simulink subsystem "saturation"  (R2024b)
settings: Solver=VariableStepAuto  StartTime=0.0  StopTime=10.0  RelTol=1e-3
settings Model: Creator=pierb  LastModifiedBy=pierb

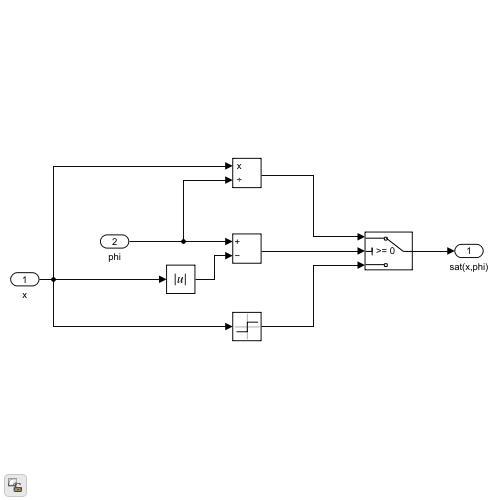
[thumbnail: Simulink's stored preview of the top-level diagram]
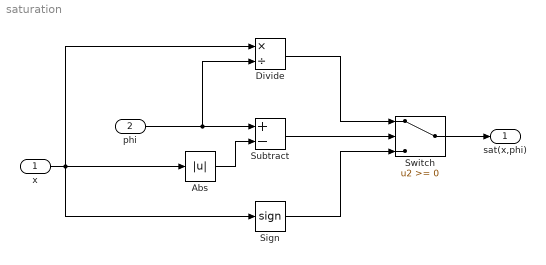
== system saturation ==
  x : Inport
  phi : Inport  Port=2
  Abs : Abs  SaturateOnIntegerOverflow=off
  Divide : Product  Inputs=*/
  Sign : Signum
  Subtract : Sum  Inputs=+-
  Switch : Switch  SaturateOnIntegerOverflow=off  InputSameDT=off
  sat(x,phi) : Outport
  wires:
  Switch/1 -> sat(x,phi)/1
  phi/1 -> Subtract/1, Divide/2
  x/1 -> Abs/1, Divide/1, Sign/1
  Abs/1 -> Subtract/2
  Subtract/1 -> Switch/2
  Divide/1 -> Switch/1
  Sign/1 -> Switch/3
